simulink model "cessna_model"  (R2025a)
settings: Solver=VariableStepAuto  StartTime=0.0  StopTime=700  RelTol=1e-3
values from neighbouring files (symbols this model uses):
  data =     [cessnadatcom.mat]
  data_ail =     [cessnadatcom.mat]
undefined symbols (not defined in the file or in its folder): m, s
libraries: aerolibasang x4, aerolibutil x3, simulink_extras x3, aerolibconvert2 x2, aerolibanim x1, aerolibadyn x1, aerolibtransform2 x1, aerolibatmos2 x1
settings Model: Creator=inigo  LastModifiedBy=inigo

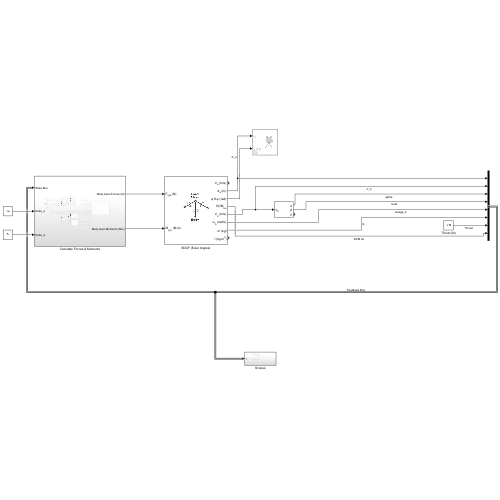
[thumbnail: Simulink's stored preview of the top-level diagram]
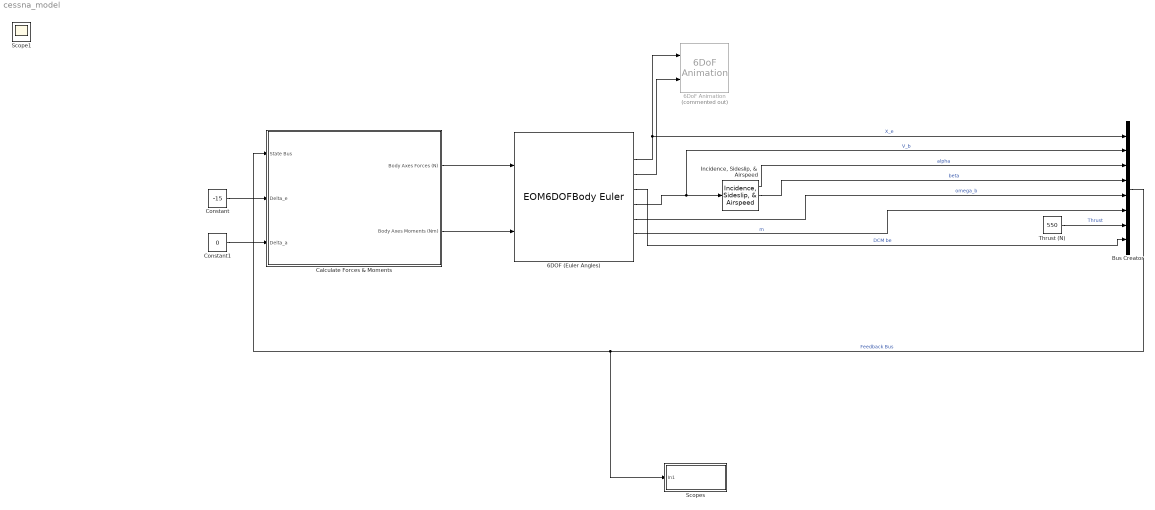
== system cessna_model ==
  6DOF (Euler Angles) : EOM6DOFBodyEuler  xme_0=[0 0 -1524]  Vm_0=[50.18 0 0]  eul_0=[0 5 0]  mass_0=1111  inertia=[1285 0 0; 0 1825 0; 0 0 2667]  mass_flag=on
  6DoF Animation : aerolibanim/6DoF Animation  Commented=on  u1=[0 4000 -2000 2000 -5000 -3000]  u2=0.1  u3=50  u4=[4000 0 -5000]  u5=Fly alongside  u6=[2000 500 -3150]  u7=10  u8=on
  Bus Creator : BusCreator  Inputs=8
  Calculate Forces & Moments : Subsystem
  Constant : Constant  Value=-15
  Constant1 : Constant  Value=0
  "Incidence, Sideslip, & Airspeed" : aerolibasang/Incidence, Sideslip, & Airspeed
  Scopes : Subsystem
  Thrust (N) : Constant  Value=550
  Scope1 : Scope
  wires:
  6DOF (Euler Angles)/5 -> Bus Creator/2, "Incidence, Sideslip, & Airspeed"/1  "V_b"
  "Incidence, Sideslip, & Airspeed"/1 -> Bus Creator/3  "alpha"
  "Incidence, Sideslip, & Airspeed"/2 -> Bus Creator/4  "beta"
  6DOF (Euler Angles)/6 -> Bus Creator/5  "omega_b"
  6DOF (Euler Angles)/3 -> 6DoF Animation/2
  Calculate Forces & Moments/1(Body Axes Forces (N)) -> 6DOF (Euler Angles)/1
  Calculate Forces & Moments/2(Body Axes Moments (Nm)) -> 6DOF (Euler Angles)/2
  6DOF (Euler Angles)/2 -> 6DoF Animation/1, Bus Creator/1  "X_e"
  6DOF (Euler Angles)/7 -> Bus Creator/6  "m"
  Bus Creator/1 -> Scopes/1(In1), Calculate Forces & Moments/1(State Bus)  "Feedback Bus"
  Thrust (N)/1 -> Bus Creator/7  "Thrust"
  6DOF (Euler Angles)/4 -> Bus Creator/8  "DCM be"
  Constant/1 -> Calculate Forces & Moments/2(Delta_e)
  Constant1/1 -> Calculate Forces & Moments/3(Delta_a)

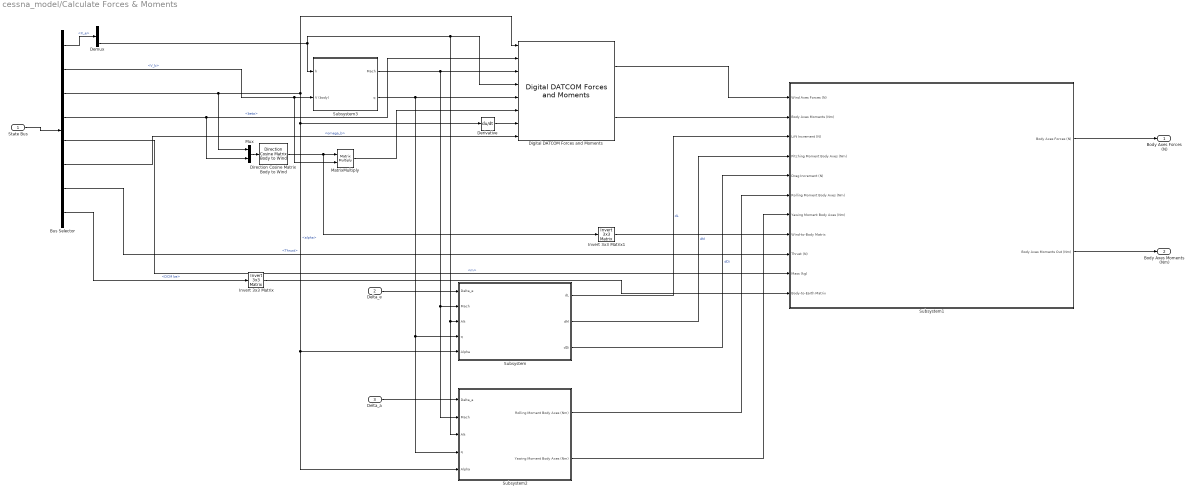
== system cessna_model/Calculate Forces & Moments ==
  State Bus : Inport
  Delta_e : Inport  Port=2
  Delta_a : Inport  Port=3
  Bus Selector : BusSelector  OutputSignals=X_e,V_b,alpha,beta,m,omega_b,Thrust,DCM be
  Demux : Demux  Outputs=3
  Derivative : Derivative
  Digital DATCOM Forces and Moments : aerolibadyn/Digital DATCOM Forces and Moments  units=Metric (MKS)  dcase=data  fmode=Wind  buildno=0  imethod=Linear  emethod=None - clip  rmethod=Clip to Range  action=Warning
  Direction Cosine Matrix Body to Wind : aerolibtransform2/Direction Cosine Matrix Body to Wind
  Invert 3x3 Matrix : aerolibutil/Invert  3x3 Matrix
  Invert 3x3 Matrix1 : aerolibutil/Invert  3x3 Matrix
  MatrixMultiply : Product  Multiplication=Matrix(*)
  Mux : Mux  Inputs=2
  Subsystem : Subsystem
  Subsystem1 : Subsystem
  Subsystem2 : Subsystem
  Subsystem3 : Subsystem
  Body Axes Forces (N) : Outport
  Body Axes Moments (Nm) : Outport  Port=2
  wires:
  State Bus/1 -> Bus Selector/1
  Subsystem3/1(Mach) -> Digital DATCOM Forces and Moments/3, Subsystem/2(Mach), Subsystem2/2(Mach)
  MatrixMultiply/1 -> Digital DATCOM Forces and Moments/6
  Subsystem3/2(q) -> Digital DATCOM Forces and Moments/5, Subsystem2/4(q), Subsystem/4(q)
  Demux/3 -> Subsystem2/3(Alt), Subsystem/3(Alt), Digital DATCOM Forces and Moments/4, Subsystem3/1(h)
  Bus Selector/1 -> Demux/1  "<X_e>"
  Bus Selector/2 -> MatrixMultiply/2, Subsystem3/2(V (body))  "<V_b>"
  Bus Selector/3 -> Mux/1, Derivative/1, Subsystem2/5(Alpha), Subsystem/5(Alpha), Digital DATCOM Forces and Moments/1  "<alpha>"
  Digital DATCOM Forces and Moments/1 -> Subsystem1/1(Wind Axes Forces (N))
  Digital DATCOM Forces and Moments/2 -> Subsystem1/2(Body Axes Moments (Nm))
  Subsystem/1(dL) -> Subsystem1/3(Lift Increment (N))  "dL"
  Subsystem/2(dM) -> Subsystem1/4(Pitching Moment Body Axes (Nm))  "dM"
  Subsystem/3(dDi) -> Subsystem1/5(Drag Increment (N))  "dDi"
  Subsystem2/1(Rolling Moment Body Axes (Nm)) -> Subsystem1/6(Rolling Moment Body Axes (Nm))
  Subsystem2/2(Yawing Moment Body Axes (Nm)) -> Subsystem1/7(Yawing Moment Body Axes (Nm))
  Bus Selector/7 -> Subsystem1/9(Thrust (N))  "<Thrust>"
  Bus Selector/4 -> Mux/2, Digital DATCOM Forces and Moments/2  "<beta>"
  Derivative/1 -> Digital DATCOM Forces and Moments/7
  Bus Selector/5 -> Subsystem1/10(Mass (kg))  "<m>"
  Bus Selector/8 -> Invert 3x3 Matrix/1  "<DCM be>"
  Invert 3x3 Matrix/1 -> Subsystem1/11(Body-to-Earth Matrix)
  Bus Selector/6 -> Digital DATCOM Forces and Moments/8  "<omega_b>"
  Direction Cosine Matrix Body to Wind/1 -> Invert 3x3 Matrix1/1, MatrixMultiply/1
  Mux/1 -> Direction Cosine Matrix Body to Wind/1
  Invert 3x3 Matrix1/1 -> Subsystem1/8(Wind-to-Body Matrix)
  Subsystem1/1(Body Axes Forces (N)) -> Body Axes Forces (N)/1
  Subsystem1/2(Body Axes Moments Out (Nm)) -> Body Axes Moments (Nm)/1
  Delta_e/1 -> Subsystem/1(Delta_e)
  Delta_a/1 -> Subsystem2/1(Delta_a)

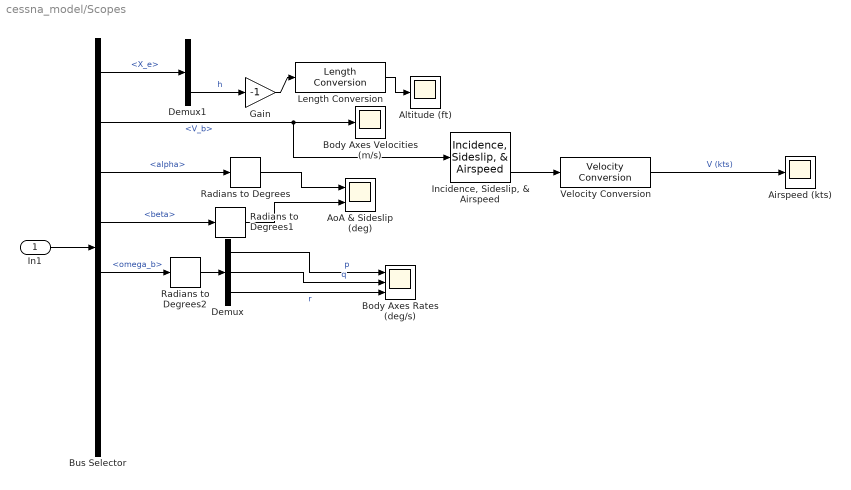
== system cessna_model/Scopes ==
  In1 : Inport
  Airspeed (kts) : Scope
      settings: ActiveDisplayYMinimum=-12.711950025121732  ActiveDisplayYMaximum=136.01057044427142  DataLoggingVariableName=ScopeData5
  Altitude (ft) : Scope
      settings: ActiveDisplayYMinimum=1268.8860961169521  ActiveDisplayYMaximum=5666.6288003006657  DataLoggingVariableName=ScopeData4
  AoA & Sideslip (deg) : Scope  NumInputPorts=2
      settings: ActiveDisplayYMinimum=-223.44306562307386  ActiveDisplayYMaximum=210.98759060767659
  Body Axes Rates (deg/s) : Scope  NumInputPorts=3
      settings: ActiveDisplayYMinimum=-177.32701709818932  ActiveDisplayYMaximum=177.65506257019479  DataLoggingVariableName=ScopeData2
  Body Axes Velocities (m/s) : Scope
      settings: ActiveDisplayYMinimum=-1  ActiveDisplayYMaximum=1  DataLoggingVariableName=ScopeData3
  Bus Selector : BusSelector  OutputSignals=X_e,V_b,alpha,beta,omega_b,m,Thrust,DCM be
  Demux : Demux  Outputs=3
  Demux1 : Demux  Outputs=3
  Gain : Gain  Gain=-1
  "Incidence, Sideslip, & Airspeed" : aerolibasang/Incidence, Sideslip, & Airspeed
  Length Conversion : aerolibconvert2/Length Conversion  IU=m  OU=ft
  Radians to Degrees : simulink_extras/Transformations/Radians to Degrees
  Radians to Degrees1 : simulink_extras/Transformations/Radians to Degrees
  Radians to Degrees2 : simulink_extras/Transformations/Radians to Degrees
  Velocity Conversion : aerolibconvert2/Velocity Conversion  IU=m/s  OU=kts
  wires:
  In1/1 -> Bus Selector/1
  Bus Selector/3 -> Radians to Degrees/1  "<alpha>"
  Bus Selector/4 -> Radians to Degrees1/1  "<beta>"
  Bus Selector/5 -> Radians to Degrees2/1  "<omega_b>"
  Demux/1 -> Body Axes Rates (deg/s)/1  "p"
  Demux/2 -> Body Axes Rates (deg/s)/2  "q"
  Demux/3 -> Body Axes Rates (deg/s)/3  "r"
  Bus Selector/2 -> "Incidence, Sideslip, & Airspeed"/1, Body Axes Velocities (m/s)/1  "<V_b>"
  Bus Selector/1 -> Demux1/1  "<X_e>"
  Demux1/3 -> Gain/1  "h"
  Gain/1 -> Length Conversion/1
  Radians to Degrees/1 -> AoA & Sideslip (deg)/1
  Radians to Degrees1/1 -> AoA & Sideslip (deg)/2
  Radians to Degrees2/1 -> Demux/1
  "Incidence, Sideslip, & Airspeed"/3 -> Velocity Conversion/1
  Velocity Conversion/1 -> Airspeed (kts)/1  "V (kts)"
  Length Conversion/1 -> Altitude (ft)/1

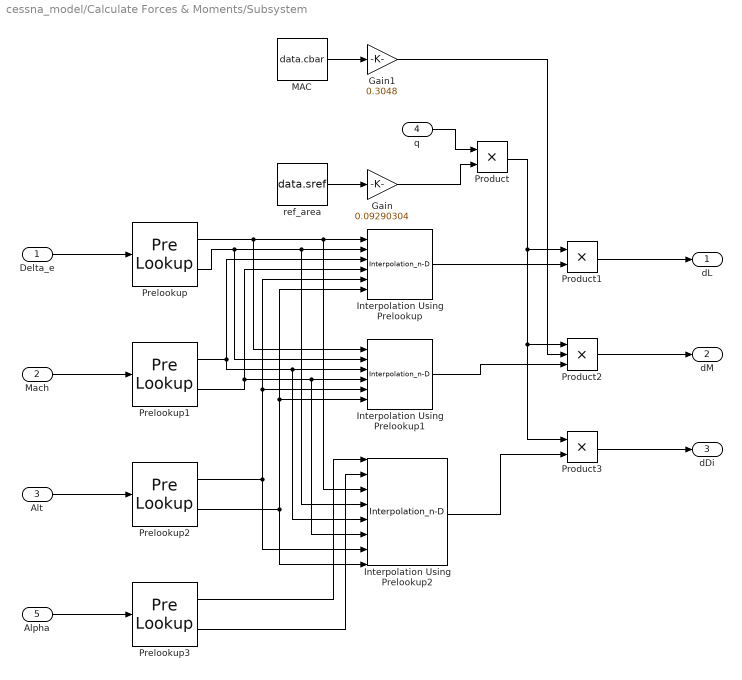
== system cessna_model/Calculate Forces & Moments/Subsystem ==
  Delta_e : Inport
  Mach : Inport  Port=2
  Alt : Inport  Port=3
  q : Inport  Port=4
  Alpha : Inport  Port=5
  Gain : Gain  Gain=0.09290304
  Gain1 : Gain  Gain=0.3048
  Interpolation Using Prelookup : Interpolation_n-D  NumberOfTableDimensions=3  Table=data.dcl_sym  InternalRulePriority=Speed
      settings: InputPortMap=u0,u1,u2,u3,u4,u5
  Interpolation Using Prelookup1 : Interpolation_n-D  NumberOfTableDimensions=3  Table=data.dcm_sym  InternalRulePriority=Speed
      settings: InputPortMap=u0,u1,u2,u3,u4,u5
  Interpolation Using Prelookup2 : Interpolation_n-D  NumberOfTableDimensions=4  Table=data.dcdi_sym  InternalRulePriority=Speed
      settings: InputPortMap=u0,u1,u2,u3,u4,u5,u6,u7
  MAC : Constant  Value=data.cbar
  Prelookup : PreLookup  BreakpointsData=data.delta  ExtrapMethod=Linear
  Prelookup1 : PreLookup  BreakpointsData=data.mach  ExtrapMethod=Linear
  Prelookup2 : PreLookup  BreakpointsData=data.alt  ExtrapMethod=Linear
  Prelookup3 : PreLookup  BreakpointsData=data.alpha  ExtrapMethod=Linear
  Product : Product
  Product1 : Product
  Product2 : Product  Inputs=3
  Product3 : Product
  ref_area : Constant  Value=data.sref
  dL : Outport
  dM : Outport  Port=2
  dDi : Outport  Port=3
  wires:
  Delta_e/1 -> Prelookup/1
  Prelookup/1 -> Interpolation Using Prelookup2/3, Interpolation Using Prelookup/1, Interpolation Using Prelookup1/1
  Prelookup/2 -> Interpolation Using Prelookup2/4, Interpolation Using Prelookup/2, Interpolation Using Prelookup1/2
  Mach/1 -> Prelookup1/1
  Prelookup1/1 -> Interpolation Using Prelookup2/5, Interpolation Using Prelookup1/3, Interpolation Using Prelookup/3
  Prelookup1/2 -> Interpolation Using Prelookup2/6, Interpolation Using Prelookup1/4, Interpolation Using Prelookup/4
  Alt/1 -> Prelookup2/1
  Prelookup2/1 -> Interpolation Using Prelookup2/7, Interpolation Using Prelookup1/5, Interpolation Using Prelookup/5
  Prelookup2/2 -> Interpolation Using Prelookup2/8, Interpolation Using Prelookup/6, Interpolation Using Prelookup1/6
  q/1 -> Product/1
  ref_area/1 -> Gain/1
  Interpolation Using Prelookup/1 -> Product1/2
  Product/1 -> Product3/1, Product2/1, Product1/1
  Interpolation Using Prelookup1/1 -> Product2/3
  Interpolation Using Prelookup2/1 -> Product3/2
  Product1/1 -> dL/1
  Product2/1 -> dM/1
  Product3/1 -> dDi/1
  Alpha/1 -> Prelookup3/1
  Prelookup3/1 -> Interpolation Using Prelookup2/1
  Prelookup3/2 -> Interpolation Using Prelookup2/2
  Gain/1 -> Product/2
  Gain1/1 -> Product2/2
  MAC/1 -> Gain1/1

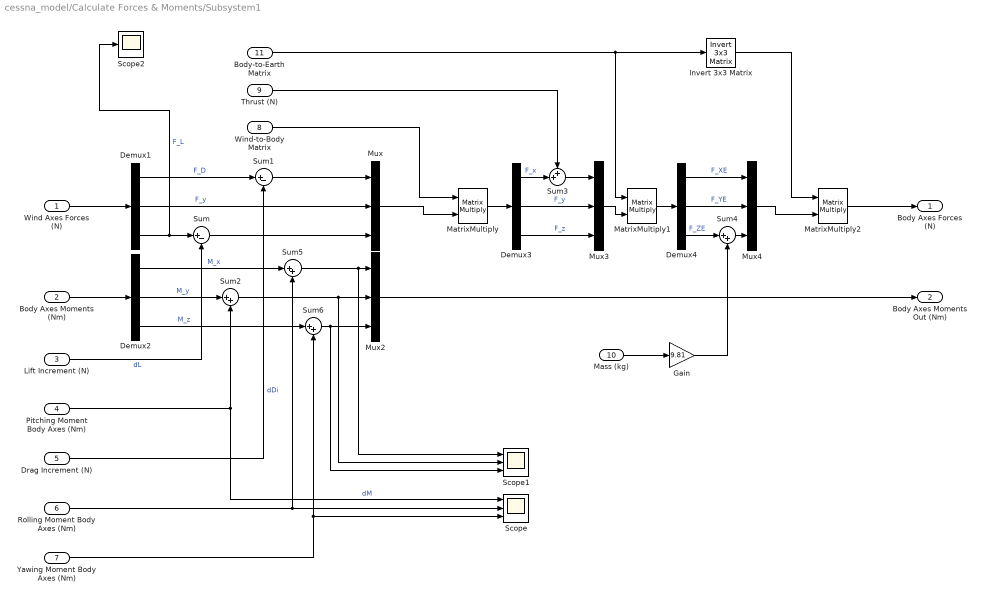
== system cessna_model/Calculate Forces & Moments/Subsystem1 ==
  Wind Axes Forces (N) : Inport
  Body Axes Moments (Nm) : Inport  Port=2
  Lift Increment (N) : Inport  Port=3
  Pitching Moment Body Axes (Nm) : Inport  Port=4
  Drag Increment (N) : Inport  Port=5
  Rolling Moment Body Axes (Nm) : Inport  Port=6
  Yawing Moment Body Axes (Nm) : Inport  Port=7
  Wind-to-Body Matrix : Inport  Port=8
  Thrust (N) : Inport  Port=9
  Mass (kg) : Inport  Port=10
  Body-to-Earth Matrix : Inport  Port=11
  Demux{1..4} (4 alike) : Demux  Outputs=3
  Gain : Gain  Gain=9.81
  Invert 3x3 Matrix : aerolibutil/Invert  3x3 Matrix
  MatrixMultiply : Product  Multiplication=Matrix(*)
  MatrixMultiply1 : Product  Multiplication=Matrix(*)
  MatrixMultiply2 : Product  Multiplication=Matrix(*)
  Mux{,2..4} (4 alike) : Mux  Inputs=3
  Scope : Scope  NumInputPorts=3
      settings: ActiveDisplayYMinimum=-1152.6742650109813  ActiveDisplayYMaximum=10374.068385098833  DataLoggingVariableName=ScopeData7
  Scope1 : Scope  NumInputPorts=3
      settings: ActiveDisplayYMinimum=-4.1091090601254047E+13  ActiveDisplayYMaximum=3.6981981528980262E+14  DataLoggingVariableName=ScopeData8
  Scope2 : Scope
      settings: ActiveDisplayYMinimum=-1  ActiveDisplayYMaximum=1  DataLoggingVariableName=ScopeData9
  Sum : Sum  Inputs=|+-
  Sum1 : Sum  Inputs=|+-
  Sum{2,4..6} (4 alike) : Sum  Inputs=|++
  Sum3 : Sum  Inputs=++|
  Body Axes Forces (N) : Outport
  Body Axes Moments Out (Nm) : Outport  Port=2
  wires:
  Mass (kg)/1 -> Gain/1
  Mux4/1 -> MatrixMultiply2/2
  Sum3/1 -> Mux3/1
  Demux3/2 -> Mux3/2  "F_y"
  MatrixMultiply/1 -> Demux3/1
  Wind-to-Body Matrix/1 -> MatrixMultiply/1
  Demux4/3 -> Sum4/1  "F_ZE"
  Mux3/1 -> MatrixMultiply1/2
  Pitching Moment Body Axes (Nm)/1 -> Scope/1, Sum2/2  "dM"
  Sum/1 -> Mux/3
  Body Axes Moments (Nm)/1 -> Demux2/1
  Demux3/3 -> Mux3/3  "F_z"
  Demux2/1 -> Sum5/1  "M_x"
  Sum4/1 -> Mux4/3
  Thrust (N)/1 -> Sum3/1
  Demux1/1 -> Sum1/1  "F_D"
  Lift Increment (N)/1 -> Sum/2  "dL"
  Demux4/2 -> Mux4/2  "F_YE"
  Body-to-Earth Matrix/1 -> Invert 3x3 Matrix/1, MatrixMultiply1/1
  Demux1/3 -> Scope2/1, Sum/1  "F_L"
  Sum2/1 -> Scope1/2, Mux2/2
  Mux2/1 -> Body Axes Moments Out (Nm)/1
  Mux/1 -> MatrixMultiply/2
  MatrixMultiply1/1 -> Demux4/1
  Demux2/2 -> Sum2/1  "M_y"
  Demux1/2 -> Mux/2  "F_y"
  Demux4/1 -> Mux4/1  "F_XE"
  Drag Increment (N)/1 -> Sum1/2  "dDi"
  Demux3/1 -> Sum3/2  "F_x"
  Sum1/1 -> Mux/1
  Wind Axes Forces (N)/1 -> Demux1/1
  Demux2/3 -> Sum6/1  "M_z"
  Gain/1 -> Sum4/2
  Invert 3x3 Matrix/1 -> MatrixMultiply2/1
  MatrixMultiply2/1 -> Body Axes Forces (N)/1
  Sum5/1 -> Scope1/1, Mux2/1
  Rolling Moment Body Axes (Nm)/1 -> Scope/2, Sum5/2
  Sum6/1 -> Scope1/3, Mux2/3
  Yawing Moment Body Axes (Nm)/1 -> Scope/3, Sum6/2

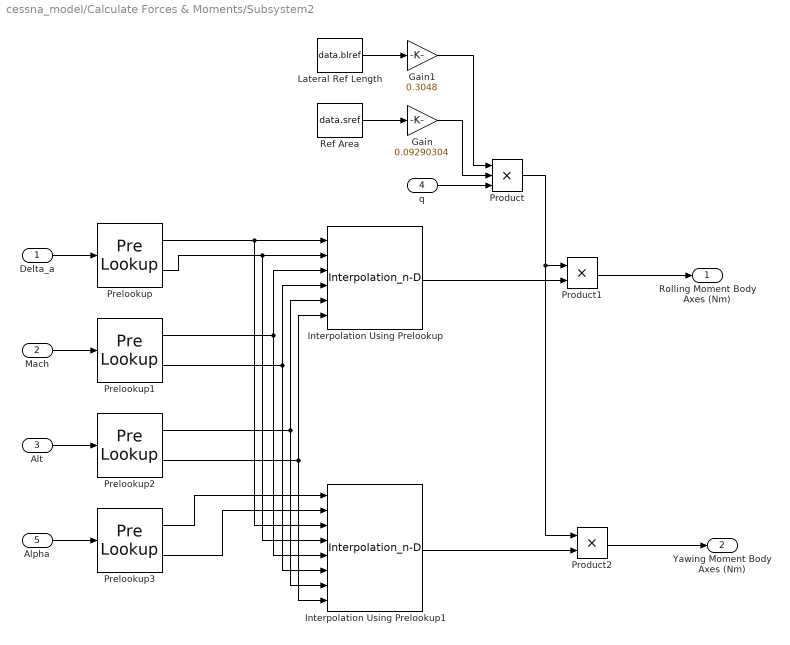
== system cessna_model/Calculate Forces & Moments/Subsystem2 ==
  Delta_a : Inport
  Mach : Inport  Port=2
  Alt : Inport  Port=3
  q : Inport  Port=4
  Alpha : Inport  Port=5
  Gain : Gain  Gain=0.09290304
  Gain1 : Gain  Gain=0.3048
  Interpolation Using Prelookup : Interpolation_n-D  NumberOfTableDimensions=3  Table=data_ail.clroll  InternalRulePriority=Speed
      settings: InputPortMap=u0,u1,u2,u3,u4,u5
  Interpolation Using Prelookup1 : Interpolation_n-D  NumberOfTableDimensions=4  Table=data_ail.cn_asy  InternalRulePriority=Speed
      settings: InputPortMap=u0,u1,u2,u3,u4,u5,u6,u7
  Lateral Ref Length : Constant  Value=data.blref
  Prelookup : PreLookup  BreakpointsData=data_ail.deltal  ExtrapMethod=Linear
  Prelookup1 : PreLookup  BreakpointsData=data_ail.mach  ExtrapMethod=Linear
  Prelookup2 : PreLookup  BreakpointsData=data_ail.alt  ExtrapMethod=Linear
  Prelookup3 : PreLookup  BreakpointsData=data_ail.alpha  ExtrapMethod=Linear
  Product : Product  Inputs=3
  Product1 : Product
  Product2 : Product
  Ref Area : Constant  Value=data.sref
  Rolling Moment Body Axes (Nm) : Outport
  Yawing Moment Body Axes (Nm) : Outport  Port=2
  wires:
  Delta_a/1 -> Prelookup/1
  Prelookup/1 -> Interpolation Using Prelookup/1, Interpolation Using Prelookup1/3
  Prelookup/2 -> Interpolation Using Prelookup/2, Interpolation Using Prelookup1/4
  Mach/1 -> Prelookup1/1
  Prelookup1/1 -> Interpolation Using Prelookup1/5, Interpolation Using Prelookup/3
  Prelookup1/2 -> Interpolation Using Prelookup1/6, Interpolation Using Prelookup/4
  Alt/1 -> Prelookup2/1
  Prelookup2/1 -> Interpolation Using Prelookup/5, Interpolation Using Prelookup1/7
  Prelookup2/2 -> Interpolation Using Prelookup/6, Interpolation Using Prelookup1/8
  Prelookup3/1 -> Interpolation Using Prelookup1/1
  Prelookup3/2 -> Interpolation Using Prelookup1/2
  Ref Area/1 -> Gain/1
  Gain/1 -> Product/2
  Interpolation Using Prelookup/1 -> Product1/2
  Product/1 -> Product2/1, Product1/1
  Product1/1 -> Rolling Moment Body Axes (Nm)/1
  Product2/1 -> Yawing Moment Body Axes (Nm)/1
  Interpolation Using Prelookup1/1 -> Product2/2
  q/1 -> Product/3
  Alpha/1 -> Prelookup3/1
  Gain1/1 -> Product/1
  Lateral Ref Length/1 -> Gain1/1

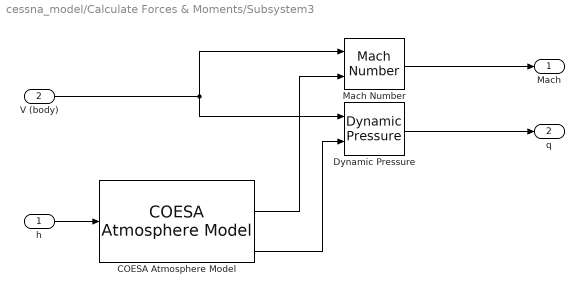
== system cessna_model/Calculate Forces & Moments/Subsystem3 ==
  h : Inport
  V (body) : Inport  Port=2
  COESA Atmosphere Model : aerolibatmos2/COESA Atmosphere Model  units=Metric (MKS)  spec=1976 COESA-extended U.S. Standard Atmosphere  model=Profile  profile_var=High temperature  profile_percent=1%  profile_alt=5 km (16404 ft)  envelope_var=High temperature  envelope_percent=1%  action=Warning
  Dynamic Pressure : aerolibasang/Dynamic Pressure
  Mach Number : aerolibasang/Mach Number
  Mach : Outport
  q : Outport  Port=2
  wires:
  h/1 -> COESA Atmosphere Model/1
  V (body)/1 -> Mach Number/1, Dynamic Pressure/1
  COESA Atmosphere Model/2 -> Mach Number/2
  COESA Atmosphere Model/4 -> Dynamic Pressure/2
  Mach Number/1 -> Mach/1
  Dynamic Pressure/1 -> q/1
